simulink subsystem "PLL"  (R2022b)
settings: Solver=VariableStepAuto  StartTime=0.0  StopTime=10.0  RelTol=1e-3
model mask{f_n=50, K_p=180, K_i=3200, df_max=50, f_c=25, theta_feedback=0, T_s=1e-4, datatype='double'}
  mask prompts: f_n "Nominal frequency [Hz]"; K_p "PI controller proportional gain"; K_i "PI controller integral gain"; df_max "Maximum detectable rate of change of frequency [Hz/s]"; f_c "Low-pass filter cutoff frequency [Hz]"; theta_feedback "Phase angle feedback (0 = external, 1 = internal)"; T_s "Sample time [s]"; datatype "Signal data type"
undefined symbols (not defined in the file or in its folder): alpha
libraries: eeGeneralControl x1, slpidlib x1, eeTransforms x1
settings Model: Creator=winkens  LastModifiedBy=winkens
settings SolverCC: AlgebraicLoopSolver=TrustRegion
settings DebuggingCC: UnconnectedInputMsg=warning  UnconnectedOutputMsg=warning  UnconnectedLineMsg=warning  SFMachineParentedDataDiag=warning
settings ModelReferenceCC: EnableRefExpFcnMdlSchedulingChecks=on
settings RTWCC: DLArmComputeVersion=19.05

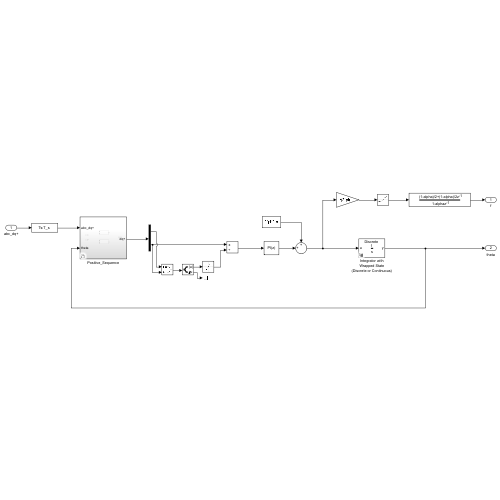
[thumbnail: Simulink's stored preview of the top-level diagram]
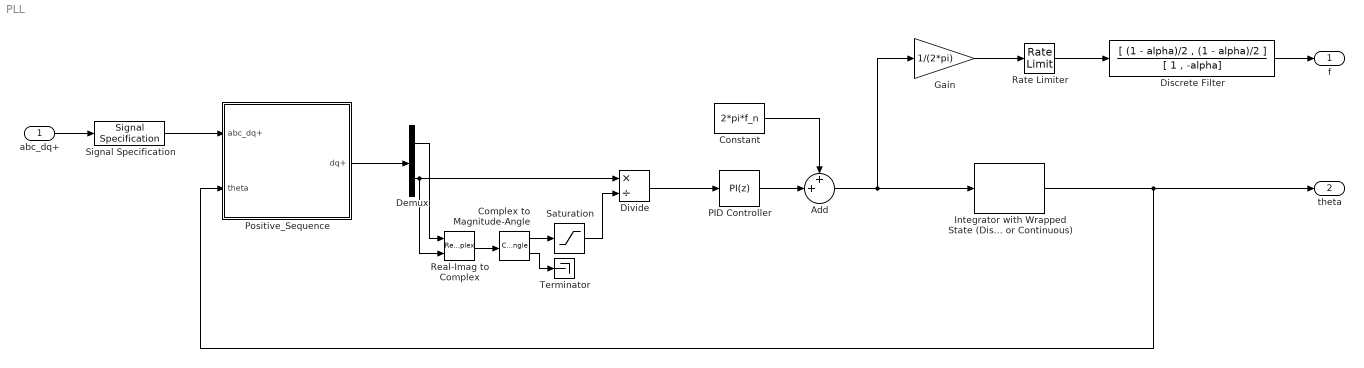
== system PLL ==
  abc_dq+ : Inport
  Add : Sum  Inputs=++|
  Complex to Magnitude-Angle : ComplexToMagnitudeAngle
  Constant : Constant  Value=2*pi*f_n  OutDataTypeStr=datatype
  Demux : Demux  Outputs=2
  Discrete Filter : DiscreteFilter  Numerator=[ (1 - alpha)/2 , (1 - alpha)/2 ]  Denominator=[ 1 , -alpha]  InitialStates=f_n  SampleTime=T_s
  Divide : Product  Inputs=*/
  Gain : Gain  Gain=1/(2*pi)
  Integrator with Wrapped State (Discrete or Continuous) : eeGeneralControl/Integrator with Wrapped State (Discrete or Continuous)  LabelModeActiveChoice=Discrete  WrappedStateUpperValue=2*pi  WrappedStateLowerValue=0  x0=0  Ts=T_s
  PID Controller : slpidlib/PID Controller  Controller=PI  Form=Parallel  TimeDomain=Discrete-time  UseExternalTs=off  SampleTime=-1  IntegratorMethod=Forward Euler  FilterMethod=Forward Euler  ControllerParametersSource=internal  P=K_p  I=K_i  UseKiTs=off  D=0  N=100  UseFilter=on  TunerSelectOption=Transfer Function Based (PID Tuner App)  InitialConditionSource=internal  InitialConditionForIntegrator=0  InitialConditionForFilter=0  DifferentiatorICPrevScaledInput=0  ExternalReset=none  TrackingMode=off  Kt=1  LimitOutput=off  SatLimitsSource=internal  UpperSaturationLimit=inf  LowerSaturationLimit=-inf  LinearizeAsGain=on  AntiWindupMode=none  Kb=1  LimitIntegrator=off  UpperIntegratorSaturationLimit=inf  LowerIntegratorSaturationLimit=-inf  POutMin=[]  POutMax=[]  IOutMin=[]  IOutMax=[]  DOutMin=[]  DOutMax=[]  NOutMin=[]  NOutMax=[]  SumOutMin=[]  SumOutMax=[]  SaturationOutMin=[]  SaturationOutMax=[]  PParamMin=[]  PParamMax=[]  IParamMin=[]  IParamMax=[]  DParamMin=[]  DParamMax=[]  NParamMin=[]  NParamMax=[]  KbParamMin=[]  KbParamMax=[]  KtParamMin=[]  KtParamMax=[]  KbOutMin=[]  KbOutMax=[]  KtOutMin=[]  KtOutMax=[]  IntegratorOutMin=[]  IntegratorOutMax=[]  FilterOutMin=[]  FilterOutMax=[]  SumI1OutMin=[]  SumI1OutMax=[]  SumI2OutMin=[]  SumI2OutMax=[]  SumI3OutMin=[]  SumI3OutMax=[]  SumI4OutMin=[]  SumI4OutMax=[]  SumDOutMin=[]  SumDOutMax=[]  DifferentiatorOutMin=[]  DifferentiatorOutMax=[]  FilterDiffOutCoefMin=[]  FilterDiffOutCoefMax=[]  ReciprocalOutMin=[]  ReciprocalOutMax=[]  SumDenOutMin=[]  SumDenOutMax=[]  SumNumOutMin=[]  SumNumOutMax=[]  DivideOutMin=[]  DivideOutMax=[]  UdiffTsProdOutMin=[]  UdiffTsProdOutMax=[]  NTsProdOutMin=[]  NTsProdOutMax=[]  UintegralTsProdOutMin=[]  UintegralTsProdOutMax=[]  UngainTsProdOutMin=[]  UngainTsProdOutMax=[]  ClampingZeroOutDataTypeStr=Inherit: Inherit via back propagation  ClampingZeroOutMin=[]  ClampingZeroOutMax=[]  FilterDenConstantOutDataTypeStr=Inherit: Inherit via back propagation  FilterDenConstantOutMin=[]  FilterDenConstantOutMax=[]  PCopyOutDataTypeStr=Inherit: Inherit via back propagation  PCopyOutMin=[]  PCopyOutMax=[]  NCopyOutDataTypeStr=Inherit: Inherit via back propagation  NCopyOutMin=[]  NCopyOutMax=[]  IntegratorContinuousStateAttributes=''  IntegratorStateMustResolveToSignalObject=off  IntegratorRTWStateStorageClass=Auto  FilterContinuousStateAttributes=''  FilterStateMustResolveToSignalObject=off  FilterRTWStateStorageClass=Auto  ParallelPVariant=InternalParameters  IdealPVariant=Disabled  IVariant=InternalParameters  DVariant=Disabled  IntegratorVariant=Discrete  SatVariant=Disabled  AWVariant=Passthrough  PCopyVariant=Disabled  TRVariant=Disabled  FdbkBlocksVariant=Forward  IdealPFdbkVariant=Disabled  SatFdbkVariant=Disabled  DerivativeFilterVariant=Disabled  NVariant=Disabled  NCopyVariant=Disabled_SignalSpec  FilterICVariant=Disabled  IntegratorICVariant=InternalICs  ExternalResetVariant=Disabled  TRSumVariant=Passthrough  SumFdbkVariant=Disabled  SumVariant=Sum_PI  TsampFilterVariant=InternalTs  TsampNgainVariant=Passthrough  TsampIntegralVariant=Passthrough  ExternalSaturationOutDataTypeStr=Inherit: Same as second input
  Positive_Sequence : Subsystem  Variant=on
  Rate Limiter : RateLimiter  RisingSlewLimit=df_max  FallingSlewLimit=-df_max  SampleTimeMode=inherited  InitialCondition=f_n
  Real-Imag to Complex : RealImagToComplex
  Saturation : Saturate  UpperLimit=inf  LowerLimit=0.1
  Signal Specification : SignalSpecification  SampleTime=T_s
  Terminator : Terminator
  f : Outport
  theta : Outport  Port=2
  wires:
  abc_dq+/1 -> Signal Specification/1
  Signal Specification/1 -> Positive_Sequence/1(abc_dq+)
  Demux/1 -> Real-Imag to Complex/1
  PID Controller/1 -> Add/2
  Constant/1 -> Add/1
  Gain/1 -> Rate Limiter/1
  Add/1 -> Integrator with Wrapped State (Discrete or Continuous)/1, Gain/1
  Integrator with Wrapped State (Discrete or Continuous)/1 -> Positive_Sequence/2(theta), theta/1
  Discrete Filter/1 -> f/1
  Rate Limiter/1 -> Discrete Filter/1
  Real-Imag to Complex/1 -> Complex to Magnitude-Angle/1
  Divide/1 -> PID Controller/1
  Demux/2 -> Divide/1, Real-Imag to Complex/2
  Complex to Magnitude-Angle/1 -> Saturation/1
  Complex to Magnitude-Angle/2 -> Terminator/1
  Saturation/1 -> Divide/2
  Positive_Sequence/1(dq+) -> Demux/1

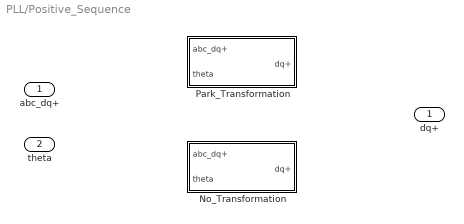
== system PLL/Positive_Sequence ==
  abc_dq+ : Inport
  theta : Inport  Port=2
  No_Transformation : Subsystem  VariantControl=theta_feedback == 0
  Park_Transformation : Subsystem  VariantControl=theta_feedback == 1
  dq+ : Outport

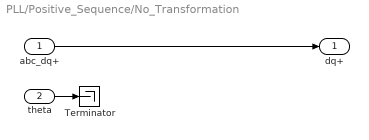
== system PLL/Positive_Sequence/No_Transformation ==
  abc_dq+ : Inport
  theta : Inport  Port=2
  Terminator : Terminator
  dq+ : Outport
  wires:
  abc_dq+/1 -> dq+/1
  theta/1 -> Terminator/1

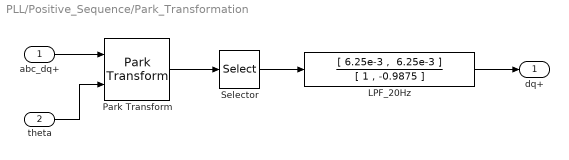
== system PLL/Positive_Sequence/Park_Transformation ==
  abc_dq+ : Inport
  theta : Inport  Port=2
  LPF_20Hz : DiscreteFilter  Numerator="[ 6.25e-3 ,  6.25e-3 ]"  Denominator=[ 1 , -0.9875 ]  SampleTime=T_s
  Park Transform : eeTransforms/Park Transform  AxisAlignment=D-axis  PowerInvariant=off
  Selector : Selector  InputPortWidth=3  IndexOptions=Index vector (dialog)  Indices=[1 2]  OutputSizes=1
  dq+ : Outport
  wires:
  abc_dq+/1 -> Park Transform/1
  theta/1 -> Park Transform/2
  Selector/1 -> LPF_20Hz/1
  Park Transform/1 -> Selector/1
  LPF_20Hz/1 -> dq+/1
